simulink model "Exp5_ANFIS_SoC_BMS"  (R2025b)
settings: Solver=FixedStepDiscrete  StartTime=0  StopTime=149  FixedStep=1  RelTol=1e-3
model workspace (MAT data in the model file):
  Exp5_I = [0 1 2 3 4 5 6 7 8 9 10 11 ... (300 elements, 150x2)]
  Exp5_SoC = [0 1 2 3 4 5 6 7 8 9 10 11 ... (300 elements, 150x2)]
  Exp5_T = [0 1 2 3 4 5 6 7 8 9 10 11 ... (300 elements, 150x2)]
  Exp5_V = [0 1 2 3 4 5 6 7 8 9 10 11 ... (300 elements, 150x2)]
  Exp5_cutoff = 5
  Exp5_fis : sugfis (value not decoded)
  Exp5_mu = [3.59237117578 0.181375030324 40.3207017989]
  Exp5_sigma = [0.347005933573 5.83790969717 11.6142704833]
  Exp5_warn = 20
libraries: simulink x2, fuzblock x1
settings Model: Creator=mithu  LastModifiedBy=mithu

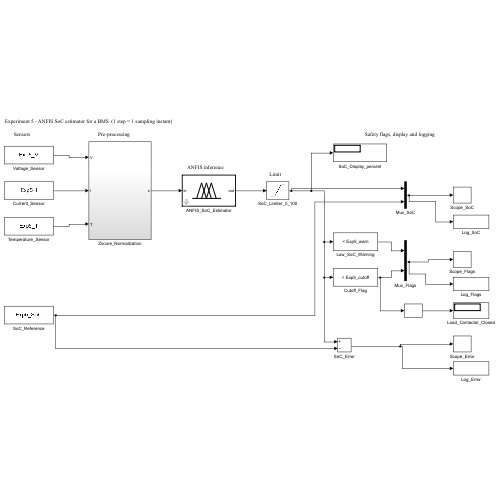
[thumbnail: Simulink's stored preview of the top-level diagram]
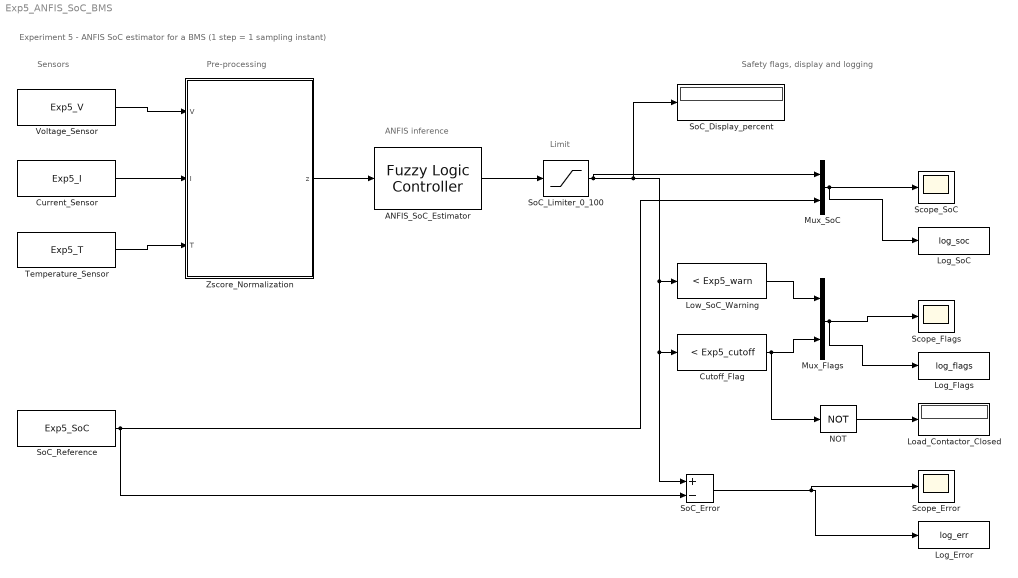
== system Exp5_ANFIS_SoC_BMS ==
  note: Experiment 5 - ANFIS SoC estimator for a BMS (1 step = 1 sampling instant)
  note: Sensors
  note: Pre-processing
  note: ANFIS inference
  note: Limit
  note: Safety flags, display and logging
  ANFIS_SoC_Estimator : fuzblock/Fuzzy Logic  Controller  FIS=Exp5_fis  OutputSampleNumber=101  DataType=double  UseLookupTable=off  NumBreakpoints=10  FuzzifiedInputs=off  RuleFiringStrengths=off  RuleOutputs=off  AggregatedOutputs=off  SimulateUsing=Interpreted execution  OutOfRangeInputValueMessage=none  NoRuleFiredMessage=none  EmptyOutputFuzzySetMessage=none
  Current_Sensor : FromWorkspace  VariableName=Exp5_I  SampleTime=1  Interpolate=off  OutputAfterFinalValue=Holding final value
  Cutoff_Flag : simulink/Logic and Bit Operations/Compare To Constant  relop=<  const=Exp5_cutoff  OutDataTypeStr=boolean
  Load_Contactor_Closed : Display
  Log_Error : ToWorkspace  VariableName=log_err  SampleTime=-1
  Log_Flags : ToWorkspace  VariableName=log_flags  SampleTime=-1
  Log_SoC : ToWorkspace  VariableName=log_soc  SampleTime=-1
  Low_SoC_Warning : simulink/Logic and Bit Operations/Compare To Constant  relop=<  const=Exp5_warn  OutDataTypeStr=boolean
  Mux_Flags : Mux  Inputs=2
  Mux_SoC : Mux  Inputs=2
  NOT : Logic  Operator=NOT  AllPortsSameDT=off  OutDataTypeStr=boolean
  Scope_Error : Scope
  Scope_Flags : Scope
  Scope_SoC : Scope
  SoC_Display_percent : Display
  SoC_Error : Sum  Inputs=+-
  SoC_Limiter_0_100 : Saturate  UpperLimit=100  LowerLimit=0
  SoC_Reference : FromWorkspace  VariableName=Exp5_SoC  SampleTime=1  Interpolate=off  OutputAfterFinalValue=Holding final value
  Temperature_Sensor : FromWorkspace  VariableName=Exp5_T  SampleTime=1  Interpolate=off  OutputAfterFinalValue=Holding final value
  Voltage_Sensor : FromWorkspace  VariableName=Exp5_V  SampleTime=1  Interpolate=off  OutputAfterFinalValue=Holding final value
  Zscore_Normalization : Subsystem
  wires:
  Voltage_Sensor/1 -> Zscore_Normalization/1(V)
  Current_Sensor/1 -> Zscore_Normalization/2(I)
  Temperature_Sensor/1 -> Zscore_Normalization/3(T)
  Zscore_Normalization/1(z) -> ANFIS_SoC_Estimator/1
  ANFIS_SoC_Estimator/1 -> SoC_Limiter_0_100/1
  SoC_Limiter_0_100/1 -> SoC_Error/1, Cutoff_Flag/1, Low_SoC_Warning/1, SoC_Display_percent/1, Mux_SoC/1
  SoC_Reference/1 -> Mux_SoC/2, SoC_Error/2
  Low_SoC_Warning/1 -> Mux_Flags/1
  Cutoff_Flag/1 -> Mux_Flags/2, NOT/1
  NOT/1 -> Load_Contactor_Closed/1
  Mux_SoC/1 -> Scope_SoC/1, Log_SoC/1
  Mux_Flags/1 -> Scope_Flags/1, Log_Flags/1
  SoC_Error/1 -> Scope_Error/1, Log_Error/1

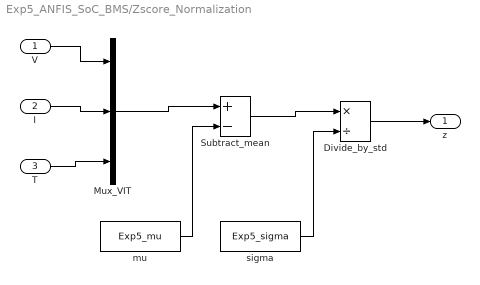
== system Exp5_ANFIS_SoC_BMS/Zscore_Normalization ==
  V : Inport
  I : Inport  Port=2
  T : Inport  Port=3
  Divide_by_std : Product  Inputs=*/
  Mux_VIT : Mux  Inputs=3
  Subtract_mean : Sum  Inputs=+-
  mu : Constant  Value=Exp5_mu
  sigma : Constant  Value=Exp5_sigma
  z : Outport
  wires:
  V/1 -> Mux_VIT/1
  I/1 -> Mux_VIT/2
  T/1 -> Mux_VIT/3
  Mux_VIT/1 -> Subtract_mean/1
  mu/1 -> Subtract_mean/2
  Subtract_mean/1 -> Divide_by_std/1
  sigma/1 -> Divide_by_std/2
  Divide_by_std/1 -> z/1
